simulink model "Controlador_LQR_ref"  (R2026a)
settings: Solver=FixedStepDiscrete  StopTime=0.05  FixedStep=Ts
InitFcn:
  | init_BOOT
values from neighbouring files (symbols this model uses):
  Ki_LQR = K_LQR(3)    [init_BOOT.m]
  Ku_LQR = K_LQR(2)    [init_BOOT.m]
  Kx_LQR = K_LQR(1)    [init_BOOT.m]
  Ts = 250e-6    (= 0.00025)    [init_BOOT.m]
undefined symbols (not defined in the file or in its folder): DiscIntNeverNeededParam
settings Model: Creator=Usuario  LastModifiedBy=Usuario
settings RTWCC: SystemTargetFile=ert.tlc  TargetLang=C++  Description=Embedded Coder
settings ERTTargetCC: RootIOFormat=Structure reference  TargetLangStandard=C++11 (ISO)  GenerateSampleERTMain=on  CodeInterfacePackaging=C++ class  SubcomponentCodeInterfacePackaging=C++ class

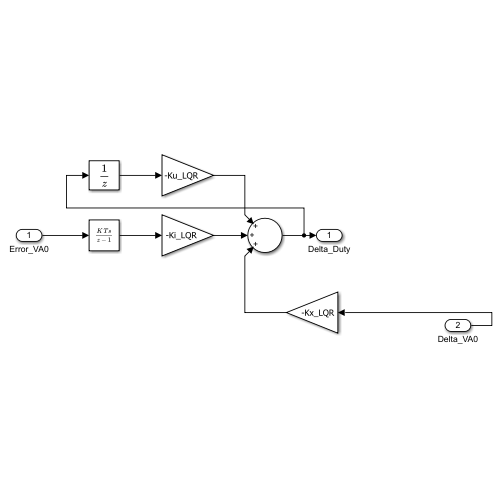
[thumbnail: Simulink's stored preview of the top-level diagram]
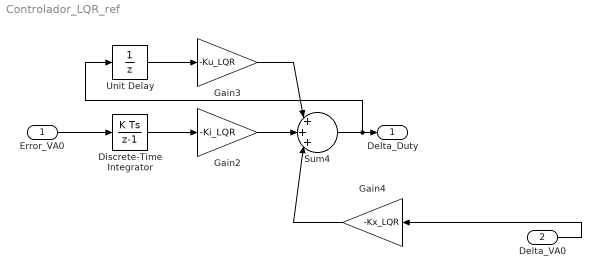
== system Controlador_LQR_ref ==
  Error_VA0 : Inport  OutDataTypeStr=double  PortDimensions=1  SampleTime=[0.00025000000000000001,0]
  Delta_VA0 : Inport  Port=2  OutDataTypeStr=double  PortDimensions=1  SampleTime=[0.00025000000000000001,0]
  Discrete-Time Integrator : DiscreteIntegrator  SampleTime=Ts  ICPrevOutput=DiscIntNeverNeededParam  ICPrevScaledInput=DiscIntNeverNeededParam
  Gain2 : Gain  Gain=-Ki_LQR
  Gain3 : Gain  Gain=-Ku_LQR
  Gain4 : Gain  Gain=-Kx_LQR
  Sum4 : Sum  Inputs=|+++|
  Unit Delay : UnitDelay  SampleTime=Ts
  Delta_Duty : Outport  OutDataTypeStr=double  PortDimensions=1  SampleTime=[0.00025000000000000001,0]
  wires:
  Unit Delay/1 -> Gain3/1
  Discrete-Time Integrator/1 -> Gain2/1
  Delta_VA0/1 -> Gain4/1
  Gain3/1 -> Sum4/1
  Gain2/1 -> Sum4/2
  Gain4/1 -> Sum4/3
  Sum4/1 -> Delta_Duty/1, Unit Delay/1
  Error_VA0/1 -> Discrete-Time Integrator/1
